simulink model "d_current_controller"  (R2025b)
settings: Solver=VariableStepAuto  StartTime=0.0  StopTime=10.0  RelTol=1e-3
undefined symbols (not defined in the file): control
settings Model: Creator=semih  LastModifiedBy=semih
settings GRTTargetCC: CombineOutputUpdateFcns=off

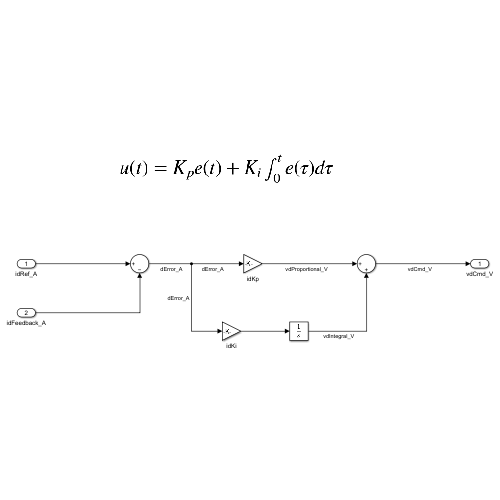
[thumbnail: Simulink's stored preview of the top-level diagram]
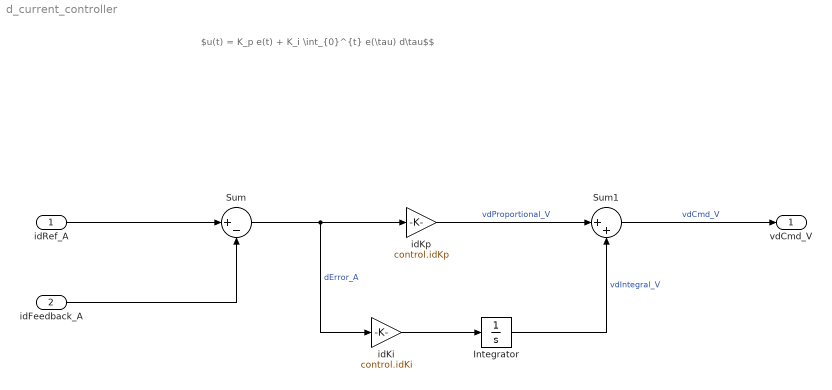
== system d_current_controller ==
  note: $u(t) = K_p e(t) + K_i \int_{0}^{t} e(\tau) d\tau$$
  idRef_A : Inport
  idFeedback_A : Inport  Port=2
  Integrator : Integrator
  Sum : Sum  Inputs=|+-
  Sum1 : Sum  Inputs=|++
  idKi : Gain  Gain=control.idKi
  idKp : Gain  Gain=control.idKp
  vdCmd_V : Outport
  wires:
  idRef_A/1 -> Sum/1
  idFeedback_A/1 -> Sum/2
  Sum/1 -> idKp/1, idKi/1  "dError_A"
  idKi/1 -> Integrator/1
  Sum1/1 -> vdCmd_V/1  "vdCmd_V"
  idKp/1 -> Sum1/1  "vdProportional_V"
  Integrator/1 -> Sum1/2  "vdIntegral_V"
